simulink library "mssSimulink"  (R2024a)
settings: Solver=ode45  StartTime=0.0  StopTime=10.0  RelTol=1e-3
undefined symbols (not defined in the file): ABC, CN_data, CX_data, CY_data, D, G, Hoerner, K_supply, kt2ms, MA, magnitude, MRB, pathlength, RAO_Amp, RAO_Dir, RAO_Freq, RAO_Phase, RAO_Vel, RAO_yaw_back, RAO_yaw_quant, RAO_yaw_quantization_flag, rho_a, slcm, T_supply, table, vessel, vesselABC
libraries: $bdroot x99, simulink x13
(part 7 of 9)

== system mssSimulink/Modelling/Kinematics/Euler angles to rotation matrix ==
  theta : Inport
  Mux : Mux  Inputs=2
  Mux2 : Mux  Inputs=9
  R11 : Fcn  Expr=u(6)*u(5)
  R12 : Fcn  Expr=u(6)*u(2)*u(1)-u(3)*u(4)
  R13 : Fcn  Expr=u(4)*u(2)*u(6)+u(3)*u(1)
  "R21 " : Fcn  Expr=u(3)*u(5)
  R22 : Fcn  Expr=u(3)*u(2)*u(1)+u(6)*u(4)
  R23 : Fcn  Expr=u(3)*u(2)*u(4)-u(6)*u(1)
  "R31 " : Fcn  Expr=-u(2)
  R32 : Fcn  Expr=u(5)*u(1)
  R33 : Fcn  Expr=u(5)*u(4)
  Reshape 9x1->3x3 : Reshape  OutputDimensionality=Customize  OutputDimensions=[3,3]
  cos(theta) : Trigonometry  Operator=cos
  sin(theta) : Trigonometry
  Rzyx : Outport  InitialOutput=0  VectorParamsAs1DForOutWhenUnconnected=off
  wires:
  R11/1 -> Mux2/1
  Mux2/1 -> Reshape 9x1->3x3/1
  Reshape 9x1->3x3/1 -> Rzyx/1
  sin(theta)/1 -> Mux/1
  cos(theta)/1 -> Mux/2
  theta/1 -> sin(theta)/1, cos(theta)/1
  Mux/1 -> R32/1, R13/1, R33/1, R23/1, R22/1, "R31 "/1, R11/1, "R21 "/1, R12/1
  R23/1 -> Mux2/8
  R13/1 -> Mux2/7
  R22/1 -> Mux2/5
  R12/1 -> Mux2/4
  "R31 "/1 -> Mux2/3
  "R21 "/1 -> Mux2/2
  R32/1 -> Mux2/6
  R33/1 -> Mux2/9

== system mssSimulink/Modelling/Kinematics/Euler angles to attitude transformation matrix ==
  theta : Inport
  Constant : Constant
  "Constant " : Constant  Value=0
  Mux2 : Mux  Inputs=9
  Reshape 9x1->3x3 : Reshape  OutputDimensionality=Customize  OutputDimensions=[3,3]
  "T21 " : Fcn  Expr=sin(u(1))*tan(u(2))
  T22 : Fcn  Expr=cos(u(1))
  T23 : Fcn  Expr=sin(u(1))/cos(u(2))
  "T31 " : Fcn  Expr=cos(u(1))*tan(u(2))
  T32 : Fcn  Expr=-sin(u(1))
  T33 : Fcn  Expr=cos(u(1))/cos(u(2))
  T : Outport  InitialOutput=0  VectorParamsAs1DForOutWhenUnconnected=off
  wires:
  Constant/1 -> Mux2/1
  Mux2/1 -> Reshape 9x1->3x3/1
  Reshape 9x1->3x3/1 -> T/1
  theta/1 -> T23/1, T33/1, T32/1, "T31 "/1, T22/1, "T21 "/1
  T23/1 -> Mux2/6
  T22/1 -> Mux2/5
  T33/1 -> Mux2/9
  "Constant "/1 -> Mux2/2, Mux2/3
  "T21 "/1 -> Mux2/4
  "T31 "/1 -> Mux2/7
  T32/1 -> Mux2/8

== system mssSimulink/Modelling/Kinematics/Rotation matrix in yaw  ==
  psi : Inport
  nu : Inport  Port=2
  Fcn : Fcn  Expr=cos(u(1))*u(2)-sin(u(1))*u(3)
  Fcn1 : Fcn  Expr=sin(u(1))*u(2)+cos(u(1))*u(3)
  Fcn2 : Fcn  Expr=u(4)
  Mux : Mux  Inputs=2
  Mux1 : Mux  Inputs=3
  R*nu : Outport  VectorParamsAs1DForOutWhenUnconnected=off
  wires:
  Mux/1 -> Fcn2/1, Fcn1/1, Fcn/1
  Fcn/1 -> Mux1/1  "x_dot"
  Fcn1/1 -> Mux1/2  "y_dot"
  Fcn2/1 -> Mux1/3  "psi_dot"
  Mux1/1 -> R*nu/1  "eta_dot"
  psi/1 -> Mux/1
  nu/1 -> Mux/2

== system mssSimulink/Modelling/Kinematics/Transformation of generalized force ==
  tau : Inport
  r_p : Inport  Port=2
  Mux : Mux  Inputs=9
  Mux1 : Mux  Inputs=2
  Product : Product  Multiplication=Matrix(*)  SaturateOnIntegerOverflow=on  OutDataTypeStr=Inherit: Same as first input
  Reshape 9x1 => 3x3 : Reshape  OutputDimensionality=Customize  OutputDimensions=[3,3]
  Selector1 : Selector  InputPortWidth=6  IndexOptions=Index vector (dialog)  Indices=[4 5 6]  OutputSizes=1
  Selector2 : Selector  InputPortWidth=6  IndexOptions=Index vector (dialog)  Indices=[1 2 3]  OutputSizes=1
  Sum : Sum  SaturateOnIntegerOverflow=on
  h11 : Fcn  Expr=0
  h12 : Fcn  Expr=u(3)
  h13 : Fcn  Expr=-u(2)
  h21 : Fcn  Expr=-u(3)
  h22 : Fcn  Expr=0
  h23 : Fcn  Expr=u(1)
  h31 : Fcn  Expr=u(2)
  h32 : Fcn  Expr=-u(1)
  h33 : Fcn  Expr=0
  inv(H'(r_p))*tau : Outport  VectorParamsAs1DForOutWhenUnconnected=off
  wires:
  tau/1 -> Selector1/1, Selector2/1
  Selector1/1 -> Sum/2  "m"
  Mux/1 -> Reshape 9x1 => 3x3/1
  Reshape 9x1 => 3x3/1 -> Product/1  "S'(r_12)"
  h11/1 -> Mux/1
  h21/1 -> Mux/2
  h31/1 -> Mux/3
  h12/1 -> Mux/4
  h22/1 -> Mux/5
  h32/1 -> Mux/6
  h13/1 -> Mux/7
  h23/1 -> Mux/8
  h33/1 -> Mux/9
  r_p/1 -> h11/1, h21/1, h31/1, h12/1, h22/1, h32/1, h13/1, h23/1, h33/1
  Mux1/1 -> inv(H'(r_p))*tau/1
  Selector2/1 -> Mux1/1, Product/2  "f"
  Sum/1 -> Mux1/2
  Product/1 -> Sum/1

== system mssSimulink/Modelling/Kinematics/Transformation of generalized velocity ==
  note: S'(r_p)
  note: omega
  note: v
  nu : Inport
  r_p : Inport  Port=2
  Mux : Mux  Inputs=9
  Mux1 : Mux  Inputs=2
  Product : Product  Multiplication=Matrix(*)  SaturateOnIntegerOverflow=on  OutDataTypeStr=Inherit: Same as first input
  Reshape 9x1 => 3x3 : Reshape  OutputDimensionality=Customize  OutputDimensions=[3,3]
  Selector1 : Selector  InputPortWidth=6  IndexOptions=Index vector (dialog)  Indices=[4 5 6]  OutputSizes=1
  Selector2 : Selector  InputPortWidth=6  IndexOptions=Index vector (dialog)  Indices=[1 2 3]  OutputSizes=1
  Sum : Sum  SaturateOnIntegerOverflow=on
  h11 : Fcn  Expr=0
  h12 : Fcn  Expr=u(3)
  h13 : Fcn  Expr=-u(2)
  h21 : Fcn  Expr=-u(3)
  h22 : Fcn  Expr=0
  h23 : Fcn  Expr=u(1)
  h31 : Fcn  Expr=u(2)
  h32 : Fcn  Expr=-u(1)
  h33 : Fcn  Expr=0
  H(r_p)*nu : Outport  VectorParamsAs1DForOutWhenUnconnected=off
  wires:
  Selector2/1 -> Sum/2
  Product/1 -> Sum/1
  Selector1/1 -> Product/2, Mux1/2
  Sum/1 -> Mux1/1
  Mux1/1 -> H(r_p)*nu/1
  r_p/1 -> h33/1, h23/1, h13/1, h32/1, h22/1, h12/1, h31/1, h21/1, h11/1
  h33/1 -> Mux/9
  h23/1 -> Mux/8
  h13/1 -> Mux/7
  h32/1 -> Mux/6
  h22/1 -> Mux/5
  h12/1 -> Mux/4
  h31/1 -> Mux/3
  h21/1 -> Mux/2
  h11/1 -> Mux/1
  Reshape 9x1 => 3x3/1 -> Product/1
  Mux/1 -> Reshape 9x1 => 3x3/1
  nu/1 -> Selector2/1, Selector1/1

== system mssSimulink/Modelling/Kinematics/Transposed rotation matrix in yaw ==
  psi : Inport
  nu : Inport  Port=2
  Mux : Mux  Inputs=2
  Mux1 : Mux  Inputs=3
  Row1 : Fcn  Expr=cos(u(1))*u(2)+sin(u(1))*u(3)
  Row2 : Fcn  Expr=-sin(u(1))*u(2)+cos(u(1))*u(3)
  Row3 : Fcn  Expr=u(4)
  Out1 : Outport  VectorParamsAs1DForOutWhenUnconnected=off
  wires:
  nu/1 -> Mux/2
  psi/1 -> Mux/1
  Mux1/1 -> Out1/1
  Row3/1 -> Mux1/3
  Row2/1 -> Mux1/2
  Row1/1 -> Mux1/1
  Mux/1 -> Row1/1, Row2/1, Row3/1

== system mssSimulink/Modelling/Kinetics /3 DOF Eqs. of motion ==
  M_RB : Inport
  M_A : Inport  Port=2
  tau : Inport  Port=3
  nu_c : Inport  Port=4
  "0 or 1   " : Gain  Gain=CoriolisOnOff-1  SaturateOnIntegerOverflow=on  OutDataTypeStr=Inherit: Same as input  ParamDataTypeStr=Inherit: Same as input
  0-1 : Gain  Gain=CoriolisOnOff  SaturateOnIntegerOverflow=on  OutDataTypeStr=Inherit: Same as input  ParamDataTypeStr=Inherit: Same as input
  3 to 6 DOF : $bdroot/Modelling/Kinetics /Support/3 to 6 DOF  SystemSampleTime=-1  VariantActivationTime=update diagram  AllowFlexibleInterface=on  Latency=0  AutoFrameSizeCalculation=off
  3 to 6 DOF1 : $bdroot/Modelling/Kinetics /Support/3 to 6 DOF  SystemSampleTime=-1  VariantActivationTime=update diagram  AllowFlexibleInterface=on  Latency=0  AutoFrameSizeCalculation=off
  6 DOF Coriolis forces : $bdroot/Modelling/Kinetics /Support/6 DOF Coriolis forces  SystemSampleTime=-1  VariantActivationTime=update diagram  AllowFlexibleInterface=on  Latency=0  AutoFrameSizeCalculation=off
  6 DOF Coriolis forces1 : $bdroot/Modelling/Kinetics /Support/6 DOF Coriolis forces  SystemSampleTime=-1  VariantActivationTime=update diagram  AllowFlexibleInterface=on  Latency=0  AutoFrameSizeCalculation=off
  6 to 3 DOF : Selector  InputPortWidth=6  IndexOptions=Index vector (dialog)  Indices=[1 2 6]  OutputSizes=1
  6 to 3 DOF1 : Selector  InputPortWidth=6  IndexOptions=Index vector (dialog)  Indices=[1 2 6]  OutputSizes=1
  Integrator1 : Integrator  InitialCondition=nu0
  Integrator2 : Integrator  InitialCondition=eta0
  M33 to M66 : $bdroot/Modelling/Kinetics /Support/M33 to M66  SystemSampleTime=-1  VariantActivationTime=update diagram  AllowFlexibleInterface=on  Latency=0  AutoFrameSizeCalculation=off
  M33 to M661 : $bdroot/Models/ Kinetics /Support/M33 to M66
  Product : Product  Inputs=/*  Multiplication=Matrix(*)  SaturateOnIntegerOverflow=on  OutDataTypeStr=Inherit: Same as first input
  "Rotation matrix in yaw " : $bdroot/Modelling/Kinematics/Rotation matrix in yaw 
  Selector2 : Selector  InputPortWidth=3  IndexOptions=Index vector (dialog)  Indices=[3]  OutputSizes=1
  Sum : Sum  Inputs=|+-  SaturateOnIntegerOverflow=on
  Sum1 : Sum  Inputs=|+-  SaturateOnIntegerOverflow=on
  Sum2 : Sum  SaturateOnIntegerOverflow=on
  Sum3 : Sum  Inputs=|+-  SaturateOnIntegerOverflow=on
  eta : Outport  VectorParamsAs1DForOutWhenUnconnected=off
  nu : Outport  Port=2  VectorParamsAs1DForOutWhenUnconnected=off
  wires:
  6 to 3 DOF1/1 -> Sum3/2
  6 to 3 DOF/1 -> Sum/2  "C_RB(nu)nu"
  6 DOF Coriolis forces1/1 -> 6 to 3 DOF1/1  "C_A(nu_r)nu_r"
  Sum3/1 -> Product/2
  Sum/1 -> Sum3/1
  3 to 6 DOF1/1 -> 6 DOF Coriolis forces1/2
  M33 to M66/1 -> 6 DOF Coriolis forces1/1
  M_A/1 -> Sum2/1, M33 to M66/1  "M_A"
  nu_c/1 -> Sum1/2
  Sum1/1 -> "0 or 1   "/1
  "0 or 1   "/1 -> 3 to 6 DOF1/1  "nu_r"
  Sum2/1 -> Product/1
  M_RB/1 -> Sum2/2, M33 to M661/1
  Integrator1/1 -> 0-1/1, Sum1/1, nu/1, "Rotation matrix in yaw "/2  "nu"
  M33 to M661/1 -> 6 DOF Coriolis forces/1
  6 DOF Coriolis forces/1 -> 6 to 3 DOF/1
  3 to 6 DOF/1 -> 6 DOF Coriolis forces/2
  0-1/1 -> 3 to 6 DOF/1
  tau/1 -> Sum/1
  Selector2/1 -> "Rotation matrix in yaw "/1  "psi"
  Integrator2/1 -> eta/1, Selector2/1  "eta"
  "Rotation matrix in yaw "/1 -> Integrator2/1  "d(eta)/dt"
  Product/1 -> Integrator1/1  "d(nu)/dt"

== system mssSimulink/Modelling/Kinetics /6 DOF Eqs. of motion ==
  M_RB : Inport
  M_A : Inport  Port=2
  tau : Inport  Port=3
  nu_c : Inport  Port=4
  0 or 1 : Gain  Gain=CoriolisOnOff-1  SaturateOnIntegerOverflow=on  OutDataTypeStr=Inherit: Same as input  ParamDataTypeStr=Inherit: Same as input
  "0 or 1   " : Gain  Gain=CoriolisOnOff-1  SaturateOnIntegerOverflow=on  OutDataTypeStr=Inherit: Same as input  ParamDataTypeStr=Inherit: Same as input
  6 DOF Coriolis forces : $bdroot/Modelling/Kinetics /Support/6 DOF Coriolis forces  SystemSampleTime=-1  VariantActivationTime=update diagram  AllowFlexibleInterface=on  Latency=0  AutoFrameSizeCalculation=off
  6 DOF Coriolis forces1 : $bdroot/Modelling/Kinetics /Support/6 DOF Coriolis forces  SystemSampleTime=-1  VariantActivationTime=update diagram  AllowFlexibleInterface=on  Latency=0  AutoFrameSizeCalculation=off
  Euler angles to rotation matrix : $bdroot/Modelling/Kinematics/Euler angles to rotation matrix
  Euler angles to attitude transformation matrix : $bdroot/Modelling/Kinematics/Euler angles to attitude transformation matrix
  Integrator : Integrator  InitialCondition=nu0
  Integrator1 : Integrator  InitialCondition=eta0(1:3)
  Integrator2 : Integrator  InitialCondition=eta0(4:6)
  Mux : Mux  Inputs=2
  Mux1 : Mux  Inputs=2
  Product : Product  Inputs=/*  Multiplication=Matrix(*)  SaturateOnIntegerOverflow=on  OutDataTypeStr=Inherit: Same as first input
  Product1 : Product  Inputs=**  Multiplication=Matrix(*)  SaturateOnIntegerOverflow=on  OutDataTypeStr=Inherit: Same as first input
  Product2 : Product  Inputs=**  Multiplication=Matrix(*)  SaturateOnIntegerOverflow=on  OutDataTypeStr=Inherit: Same as first input
  Selector1 : Selector  InputPortWidth=6  IndexOptions=Index vector (dialog)  Indices=[1 2 3]  OutputSizes=1
  Selector2 : Selector  InputPortWidth=6  IndexOptions=Index vector (dialog)  Indices=[4 5 6]  OutputSizes=1
  Sum : Sum  Inputs=|+-  SaturateOnIntegerOverflow=on
  Sum1 : Sum  Inputs=|+-  SaturateOnIntegerOverflow=on
  Sum2 : Sum  SaturateOnIntegerOverflow=on
  Sum3 : Sum  Inputs=|+-  SaturateOnIntegerOverflow=on
  eta : Outport  VectorParamsAs1DForOutWhenUnconnected=off
  nu : Outport  Port=2  VectorParamsAs1DForOutWhenUnconnected=off
  wires:
  nu_c/1 -> Sum1/2
  Sum1/1 -> "0 or 1   "/1
  "0 or 1   "/1 -> 6 DOF Coriolis forces1/2  "nu_r"
  6 DOF Coriolis forces1/1 -> Sum3/2  "C_A(nu_r)nu_r"
  Sum3/1 -> Product/2
  Sum/1 -> Sum3/1
  Sum2/1 -> Product/1  "M"
  M_A/1 -> Sum2/1, 6 DOF Coriolis forces1/1  "M_A"
  M_RB/1 -> Sum2/2, 6 DOF Coriolis forces/1  "M_RB"
  Product/1 -> Integrator/1  "(d/dt)nu"
  Integrator/1 -> Selector1/1, Selector2/1, 0 or 1/1  "nu"
  Selector1/1 -> Product1/2, Mux1/1  "v"
  Selector2/1 -> Mux1/2, Product2/2  "w_nb"
  Product1/1 -> Integrator1/1  "dp/dt"
  Euler angles to rotation matrix/1 -> Product1/1  "R(theta)"
  Product2/1 -> Integrator2/1  "(d/dt)theta"
  Integrator2/1 -> Mux/2, Euler angles to rotation matrix/1, Euler angles to attitude transformation matrix/1  "theta"
  Integrator1/1 -> Mux/1  "p"
  Mux/1 -> eta/1  "eta"
  Mux1/1 -> Sum1/1, nu/1  "nu"
  Euler angles to attitude transformation matrix/1 -> Product2/1
  tau/1 -> Sum/1
  6 DOF Coriolis forces/1 -> Sum/2  "C_RB(nu)nu"
  0 or 1/1 -> 6 DOF Coriolis forces/2

== system mssSimulink/Modelling/Kinetics /Support ==
  3 to 6 DOF : Subsystem
      mask Display: disp('modes,\n 1,2,6, to\n 6 DOF')
  4 to 6 DOF : Subsystem
      mask Display: disp('modes,\n 1,2,4,6, to\n 6 DOF')
  6 DOF Coriolis forces : Subsystem
  6 to 3 DOF : Selector  InputPortWidth=6  IndexOptions=Index vector (dialog)  Indices=[1 2 6]  OutputSizes=1
  6 to 4 DOF : Selector  InputPortWidth=6  IndexOptions=Index vector (dialog)  Indices=[1 2 4 6]  OutputSizes=1
  M33 to M66 : Subsystem
      mask Display: disp('add zeros')
  M44 to M66 : Subsystem
      mask Display: disp('add zeros')
  M66 to M33 : Selector  NumberOfDimensions=2  InputPortWidth=3  IndexOptions=Index vector (dialog),Index vector (dialog)  Indices=[1 2 6],[1 2 6]  OutputSizes=1
  M66 to M44 : Selector  NumberOfDimensions=2  InputPortWidth=3  IndexOptions=Index vector (dialog),Index vector (dialog)  Indices=[1 2 4 6],[1 2 4 6]  OutputSizes=1

== system mssSimulink/Modelling/Propulsion/Actuator Configuration ==
  2 main propellers and 3 tunnel  thrusters : Subsystem
      mask Display: disp('tau = T*K(n)*u')
  "2 main propellers, 1 azimuth and 2 tunnel thrusters" : Subsystem
      mask Display:
      | disp('tau =            \n\n')
      | disp('    T(alpha)*K(n)*u')
  4 azimuth thrusters : Subsystem
      mask Display:
      | disp('tau =            \n\n')
      | disp('    T(alpha)*K(n)*u')
  Column vector t : Subsystem
  Thruster configuration matrix : Subsystem

== system mssSimulink/Modelling/Propulsion/Open-water propeller characteristics ==
  n : Inport
  Va : Inport  Port=2
  Dot Product1 : DotProduct  OutDataTypeStr=Inherit: Inherit via internal rule
  Dot Product2 : DotProduct  OutDataTypeStr=Inherit: Inherit via internal rule
  Kq poly : Constant  Value=Par_Thruster_Kqp
  Kt poly : Constant  Value=Par_Thruster_Ktp
  Math Function3 : Math  Operator=magnitude^2  SignedPower=on
  Math Function4 : Math  Operator=magnitude^2  SignedPower=on
  Mux1 : Mux  Inputs=3
  Product{2..3,6,9..10} (5 alike) : Product  SaturateOnIntegerOverflow=on  OutDataTypeStr=Inherit: Same as first input
  Sign : Signum
  Switch : Switch  InputSameDT=off
  Zero limit : Saturate  UpperLimit=inf  LowerLimit=0
  Zero limit1 : Saturate  UpperLimit=inf  LowerLimit=0
  Zero limit2 : Saturate  UpperLimit=inf  LowerLimit=0
  reverse reduction : Gain  Gain=Par_Thruster_reverse_reduction  SaturateOnIntegerOverflow=on  OutDataTypeStr=Inherit: Same as input  ParamDataTypeStr=Inherit: Same as input
  rhow[D^2 D^3 D^4] : Constant  Value=Glob_rhow*[Par_Thruster_D^2 Par_Thruster_D^3 Par_Thruster_D^4]
  "rhow[D^3 D^4 D^5] " : Constant  Value=Glob_rhow*[Par_Thruster_D^3 Par_Thruster_D^4 Par_Thruster_D^5]
  T_a : Outport  VectorParamsAs1DForOutWhenUnconnected=off
  Q_a : Outport  Port=2  VectorParamsAs1DForOutWhenUnconnected=off
  wires:
  Product10/1 -> Mux1/2
  Math Function4/1 -> Mux1/3
  Math Function3/1 -> Mux1/1
  n/1 -> Sign/1, Product10/2, Math Function4/1
  Product9/1 -> Dot Product2/2
  "rhow[D^3 D^4 D^5] "/1 -> Product9/2
  Kq poly/1 -> Product9/1
  Product6/1 -> Dot Product1/1
  rhow[D^2 D^3 D^4]/1 -> Product6/2
  Kt poly/1 -> Product6/1
  Sign/1 -> Product3/2, Switch/2, Product2/2
  Va/1 -> Zero limit2/1
  Zero limit1/1 -> Product3/1
  Zero limit/1 -> Product2/1
  Dot Product2/1 -> Zero limit1/1
  Dot Product1/1 -> Zero limit/1
  Product3/1 -> Q_a/1
  Product2/1 -> Switch/1, reverse reduction/1
  Switch/1 -> T_a/1
  reverse reduction/1 -> Switch/3
  Mux1/1 -> Dot Product2/1, Dot Product1/2
  Zero limit2/1 -> Math Function3/1, Product10/1

== system mssSimulink/Modelling/Propulsion/Propeller shaft dynamics ==
  RPM_c : Inport
  Gain : Gain  Gain=1/tc  SaturateOnIntegerOverflow=on  OutDataTypeStr=Inherit: Same as input  ParamDataTypeStr=Inherit: Same as input
  Integrator1 : Integrator
  Saturation : Saturate  UpperLimit=rpm_rate  LowerLimit=-rpm_rate
  Saturation1 : Saturate  UpperLimit=rpm_max  LowerLimit=-rpm_max
  Sum1 : Sum  Inputs=|+-  InputSameDT=on  SaturateOnIntegerOverflow=on  OutDataTypeStr=Inherit: Same as first input
  RPM : Outport  VectorParamsAs1DForOutWhenUnconnected=off
  wires:
  RPM_c/1 -> Saturation1/1
  Saturation/1 -> Integrator1/1
  Saturation1/1 -> Sum1/1
  Integrator1/1 -> Sum1/2, RPM/1
  Sum1/1 -> Gain/1
  Gain/1 -> Saturation/1

== system mssSimulink/Navigation/Estimators/Discerte-time EKF for SOG and COG ==
  xpos : Inport
  ypos : Inport  Port=2
  Five-state EKF for North-East positions : MATLAB Function  InitFcn=clear EKF_5states;  TreatAsAtomicUnit=on
  Qd : Constant  Value=Qd
  RT : RateTransition  OutPortSampleTime=0
  Rate Transition : RateTransition  OutPortSampleTimeMultiple=10  OutPortSampleTime=h_samp
  Rate Transition1 : RateTransition  OutPortSampleTimeMultiple=10  OutPortSampleTime=h_samp
  Rd : Constant  Value=Rd
  alpha_1 : Constant  Value=alpha_1
  alpha_2 : Constant  Value=alpha_2
  h_samp : Constant  Value=h_samp
  x_hat : Outport
  wires:
  RT/1 -> x_hat/1
  xpos/1 -> Rate Transition/1
  ypos/1 -> Rate Transition1/1
  h_samp/1 -> Five-state EKF for North-East positions/3(h_samp)
  Five-state EKF for North-East positions/1(x_hat) -> RT/1
  Rate Transition/1 -> Five-state EKF for North-East positions/1(position1)
  Rate Transition1/1 -> Five-state EKF for North-East positions/2(position2)
  Qd/1 -> Five-state EKF for North-East positions/4(Qd)
  Rd/1 -> Five-state EKF for North-East positions/5(Rd)
  alpha_1/1 -> Five-state EKF for North-East positions/6(alpha_1)
  alpha_2/1 -> Five-state EKF for North-East positions/7(alpha_2)

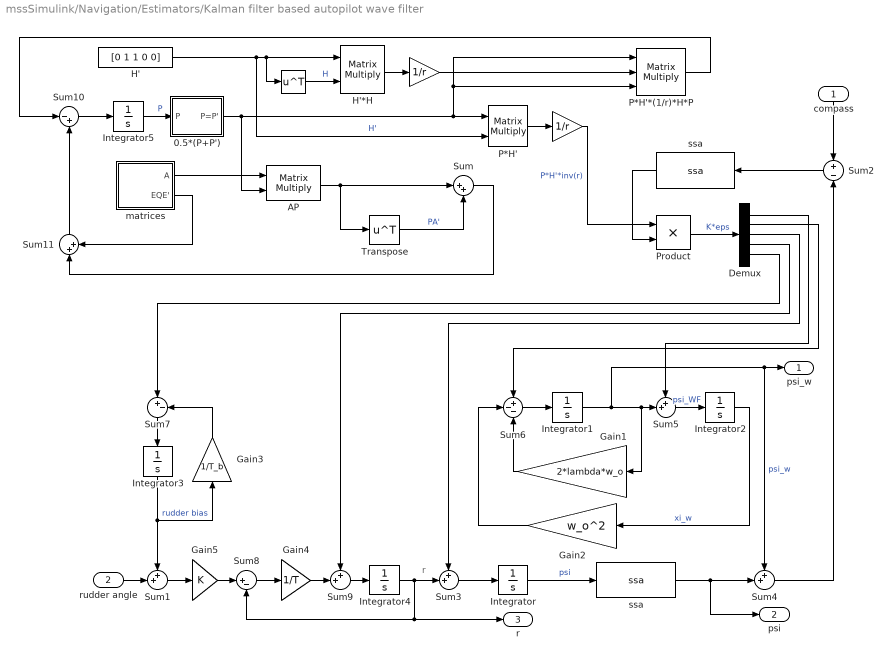
== system mssSimulink/Navigation/Estimators/Kalman filter based autopilot wave filter ==
  note: r
  compass : Inport
  rudder angle : Inport  Port=2
  "  " : Math  Operator=transpose  SignedPower=on
  "    " : Gain  Gain=1/r  SaturateOnIntegerOverflow=on  OutDataTypeStr=Inherit: Same as input  ParamDataTypeStr=Inherit: Same as input
  "     " : Gain  Gain=1/r  SaturateOnIntegerOverflow=on  OutDataTypeStr=Inherit: Same as input  ParamDataTypeStr=Inherit: Same as input
  0.5*(P+P') : Subsystem
  AP : Product  Multiplication=Matrix(*)  SaturateOnIntegerOverflow=on  OutDataTypeStr=Inherit: Same as first input
  Demux : Demux  Outputs=5
      settings: DisplayOption=none
  Gain1 : Gain  Gain=2*lambda*w_o  SaturateOnIntegerOverflow=on  OutDataTypeStr=Inherit: Same as input  ParamDataTypeStr=Inherit: Same as input
  Gain2 : Gain  Gain=w_o^2  SaturateOnIntegerOverflow=on  OutDataTypeStr=Inherit: Same as input  ParamDataTypeStr=Inherit: Same as input
  Gain3 : Gain  Gain=1/T_b  SaturateOnIntegerOverflow=on  OutDataTypeStr=Inherit: Same as input  ParamDataTypeStr=Inherit: Same as input
  Gain4 : Gain  Gain=1/T  SaturateOnIntegerOverflow=on  OutDataTypeStr=Inherit: Same as input  ParamDataTypeStr=Inherit: Same as input
  Gain5 : Gain  Gain=K  SaturateOnIntegerOverflow=on  OutDataTypeStr=Inherit: Same as input  ParamDataTypeStr=Inherit: Same as input
  H' : Constant  Value=[0 1 1 0 0]
  H'*H : Product  Multiplication=Matrix(*)  SaturateOnIntegerOverflow=on  OutDataTypeStr=Inherit: Same as first input
  Integrator{,1..4} (5 alike) : Integrator
  Integrator5 : Integrator  InitialCondition=P0
  P*H' : Product  Inputs=**  Multiplication=Matrix(*)  SaturateOnIntegerOverflow=on  OutDataTypeStr=Inherit: Same as first input
  P*H'*(1/r)*H*P : Product  Inputs=***  Multiplication=Matrix(*)  SaturateOnIntegerOverflow=on  OutDataTypeStr=Inherit: Same as first input
  Product : Product  SaturateOnIntegerOverflow=on  OutDataTypeStr=Inherit: Same as first input
  Sum : Sum  Inputs=|++  SaturateOnIntegerOverflow=on
  Sum{1,3..5,9} (5 alike) : Sum  Inputs=++|  InputSameDT=on  SaturateOnIntegerOverflow=on  OutDataTypeStr=Inherit: Same as first input
  Sum10 : Sum  Inputs=|-+  SaturateOnIntegerOverflow=on
  Sum11 : Sum  Inputs=|++  SaturateOnIntegerOverflow=on
  Sum2 : Sum  Inputs=+|-  InputSameDT=on  SaturateOnIntegerOverflow=on  OutDataTypeStr=Inherit: Same as first input
  Sum6 : Sum  Inputs=+--  InputSameDT=on  SaturateOnIntegerOverflow=on  OutDataTypeStr=Inherit: Same as first input
  Sum7 : Sum  Inputs=|+-  InputSameDT=on  SaturateOnIntegerOverflow=on  OutDataTypeStr=Inherit: Same as first input
  Sum8 : Sum  Inputs=|+-  InputSameDT=on  SaturateOnIntegerOverflow=on  OutDataTypeStr=Inherit: Same as first input
  Transpose : Math  Operator=transpose  SignedPower=on
  matrices : Subsystem
  "ssa " : $bdroot/Utilities/Math Operations/ssa  SystemSampleTime=-1  VariantActivationTime=update diagram  AllowFlexibleInterface=on  Latency=0  AutoFrameSizeCalculation=off
  "ssa  " : $bdroot/Utilities/Math Operations/ssa  SystemSampleTime=-1  VariantActivationTime=update diagram  AllowFlexibleInterface=on  Latency=0  AutoFrameSizeCalculation=off
  psi_w : Outport  VectorParamsAs1DForOutWhenUnconnected=off
  psi : Outport  Port=2  VectorParamsAs1DForOutWhenUnconnected=off
  r : Outport  Port=3  VectorParamsAs1DForOutWhenUnconnected=off
  wires:
  0.5*(P+P')/1(P=P') -> P*H'*(1/r)*H*P/1, P*H'*(1/r)*H*P/3, P*H'/1, AP/2
  Integrator5/1 -> 0.5*(P+P')/1(P)  "P"
  P*H'*(1/r)*H*P/1 -> Sum10/1
  Demux/4 -> Sum9/1
  Demux/3 -> Sum3/1
  Demux/2 -> Sum6/1
  Demux/1 -> Sum5/1
  Product/1 -> Demux/1  "K*eps"
  "ssa "/1 -> Product/2
  Sum/1 -> Sum11/1
  matrices/2(EQE') -> Sum11/2
  "     "/1 -> Product/1  "P*H'*inv(r)"
  Sum11/1 -> Sum10/2
  Transpose/1 -> Sum/2  "PA'"
  Sum10/1 -> Integrator5/1
  AP/1 -> Transpose/1, Sum/1
  Sum9/1 -> Integrator4/1
  Gain4/1 -> Sum9/2
  Gain5/1 -> Sum8/1
  Gain3/1 -> Sum7/2
  Integrator3/1 -> Gain3/1, Sum1/1  "rudder bias"
  Sum7/1 -> Integrator3/1
  Demux/5 -> Sum7/1
  Integrator4/1 -> Sum3/2, r/1, Sum8/2
  Sum8/1 -> Gain4/1
  rudder angle/1 -> Sum1/2
  compass/1 -> Sum2/1
  Sum1/1 -> Gain5/1
  Integrator1/1 -> psi_w/1, Sum4/1, Gain1/1, Sum5/2  "psi_w"
  Sum5/1 -> Integrator2/1  "psi_WF"
  Integrator2/1 -> Gain2/1  "xi_w"
  Gain2/1 -> Sum6/2
  Gain1/1 -> Sum6/3
  Sum6/1 -> Integrator1/1
  Sum4/1 -> Sum2/2
  "ssa  "/1 -> psi/1, Sum4/2
  Integrator/1 -> "ssa  "/1  "psi"
  Sum2/1 -> "ssa "/1
  Sum3/1 -> Integrator/1
  H'/1 -> "  "/1, H'*H/1, P*H'/2  "H'"
  H'*H/1 -> "    "/1
  P*H'/1 -> "     "/1
  "    "/1 -> P*H'*(1/r)*H*P/2
  "  "/1 -> H'*H/2  "H"
  matrices/1(A) -> AP/1

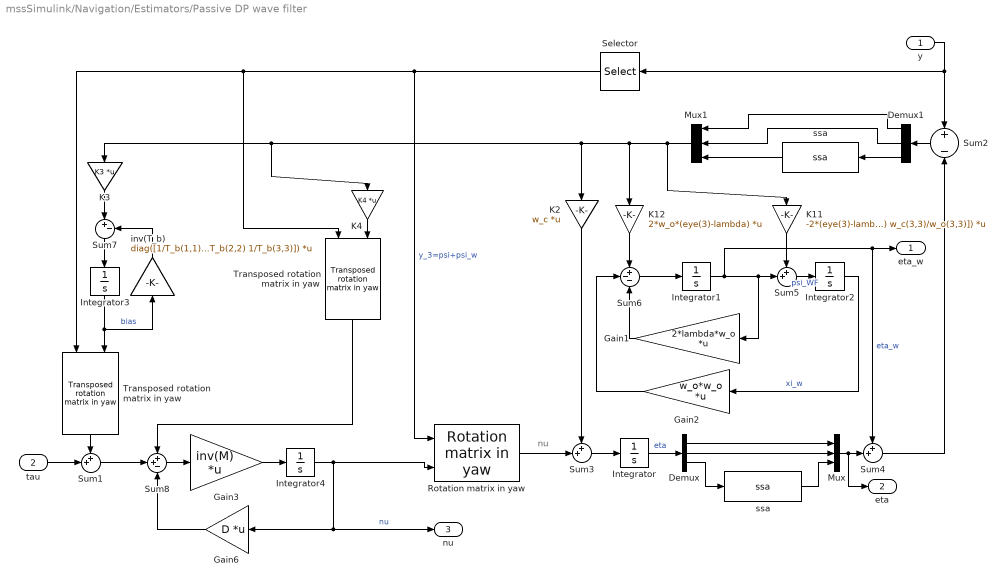
== system mssSimulink/Navigation/Estimators/Passive DP wave filter ==
  note: nu
  y : Inport
  tau : Inport  Port=2
  Demux : Demux  Outputs=3
      settings: DisplayOption=none
  Demux1 : Demux  Outputs=3
      settings: DisplayOption=none
  Gain1 : Gain  Gain=2*lambda*w_o  Multiplication=Matrix(K*u)  SaturateOnIntegerOverflow=on  OutDataTypeStr=Inherit: Same as input  ParamDataTypeStr=Inherit: Same as input
  Gain2 : Gain  Gain=w_o*w_o  Multiplication=Matrix(K*u)  SaturateOnIntegerOverflow=on  OutDataTypeStr=Inherit: Same as input  ParamDataTypeStr=Inherit: Same as input
  Gain3 : Gain  Gain=inv(M)  Multiplication=Matrix(K*u)  SaturateOnIntegerOverflow=on  OutDataTypeStr=Inherit: Same as input  ParamDataTypeStr=Inherit: Same as input
  Gain6 : Gain  Gain=D  Multiplication=Matrix(K*u)  SaturateOnIntegerOverflow=on  OutDataTypeStr=Inherit: Same as input  ParamDataTypeStr=Inherit: Same as input
  Integrator{,1..4} (5 alike) : Integrator
  K11 : Gain  Gain=-2*(eye(3)-lambda)*diag([w_c(1,1)/w_o(1,1) w_c(2,2)/w_o(2,2) w_c(3,3)/w_o(3,3)])  Multiplication=Matrix(K*u)  SaturateOnIntegerOverflow=on  OutDataTypeStr=Inherit: Same as input  ParamDataTypeStr=Inherit: Same as input
  K12 : Gain  Gain=2*w_o*(eye(3)-lambda)  Multiplication=Matrix(K*u)  SaturateOnIntegerOverflow=on  OutDataTypeStr=Inherit: Same as input  ParamDataTypeStr=Inherit: Same as input
  K2 : Gain  Gain=w_c  Multiplication=Matrix(K*u)  SaturateOnIntegerOverflow=on  OutDataTypeStr=Inherit: Same as input  ParamDataTypeStr=Inherit: Same as input
  K3 : Gain  Gain=K3  Multiplication=Matrix(K*u)  SaturateOnIntegerOverflow=on  OutDataTypeStr=Inherit: Same as input  ParamDataTypeStr=Inherit: Same as input
  K4 : Gain  Gain=K4  Multiplication=Matrix(K*u)  SaturateOnIntegerOverflow=on  OutDataTypeStr=Inherit: Same as input  ParamDataTypeStr=Inherit: Same as input
  Mux : Mux  Inputs=3
  Mux1 : Mux  Inputs=3
  "Rotation matrix in yaw   " : $bdroot/Modelling/Kinematics/Rotation matrix in yaw 
  Selector : Selector  InputPortWidth=3  IndexOptions=Index vector (dialog)  Indices=[3]  OutputSizes=1
  Sum{1,3..5} (4 alike) : Sum  Inputs=++|  InputSameDT=on  SaturateOnIntegerOverflow=on  OutDataTypeStr=Inherit: Same as first input
  Sum2 : Sum  Inputs=+|-  InputSameDT=on  SaturateOnIntegerOverflow=on  OutDataTypeStr=Inherit: Same as first input
  Sum6 : Sum  Inputs=+--  InputSameDT=on  SaturateOnIntegerOverflow=on  OutDataTypeStr=Inherit: Same as first input
  Sum7 : Sum  Inputs=|+-  InputSameDT=on  SaturateOnIntegerOverflow=on  OutDataTypeStr=Inherit: Same as first input
  Sum8 : Sum  Inputs=++-  InputSameDT=on  SaturateOnIntegerOverflow=on  OutDataTypeStr=Inherit: Same as first input
  "Transposed rotation matrix in yaw " : $bdroot/Modelling/Kinematics/Transposed rotation  matrix in yaw
  "Transposed rotation matrix in yaw     " : $bdroot/Modelling/Kinematics/Transposed rotation  matrix in yaw
  inv(T_b) : Gain  Gain=diag([1/T_b(1,1) 1/T_b(2,2) 1/T_b(3,3)])  Multiplication=Matrix(K*u)  SaturateOnIntegerOverflow=on  OutDataTypeStr=Inherit: Same as input  ParamDataTypeStr=Inherit: Same as input
  "ssa " : $bdroot/Utilities/Math Operations/ssa  SystemSampleTime=-1  VariantActivationTime=update diagram  AllowFlexibleInterface=on  Latency=0  AutoFrameSizeCalculation=off
  "ssa   " : $bdroot/Utilities/Math Operations/ssa  SystemSampleTime=-1  VariantActivationTime=update diagram  AllowFlexibleInterface=on  Latency=0  AutoFrameSizeCalculation=off
  eta_w : Outport  VectorParamsAs1DForOutWhenUnconnected=off
  eta : Outport  Port=2  VectorParamsAs1DForOutWhenUnconnected=off
  nu : Outport  Port=3  VectorParamsAs1DForOutWhenUnconnected=off
  wires:
  Sum3/1 -> Integrator/1
  Mux1/1 -> K11/1, K12/1, K2/1, K3/1, K4/1
  Sum4/1 -> Sum2/2
  K2/1 -> Sum3/1
  Sum6/1 -> Integrator1/1
  Gain1/1 -> Sum6/3
  Gain2/1 -> Sum6/2
  Integrator2/1 -> Gain2/1  "xi_w"
  K11/1 -> Sum5/1
  K12/1 -> Sum6/1
  Sum5/1 -> Integrator2/1  "psi_WF"
  Integrator1/1 -> Sum5/2, Gain1/1, Sum4/1, eta_w/1  "eta_w"
  y/1 -> Sum2/1, Selector/1
  tau/1 -> Sum1/2
  Sum7/1 -> Integrator3/1
  Integrator3/1 -> inv(T_b)/1, "Transposed rotation matrix in yaw "/2  "bias"
  inv(T_b)/1 -> Sum7/2
  Integrator/1 -> Demux/1  "eta"
  "ssa "/1 -> Mux/3
  Mux/1 -> Sum4/2, eta/1
  Demux/1 -> Mux/1
  Demux/2 -> Mux/2
  "ssa   "/1 -> Mux1/3
  Demux1/2 -> Mux1/2
  Demux1/3 -> "ssa   "/1
  Sum2/1 -> Demux1/1
  Demux1/1 -> Mux1/1
  Selector/1 -> "Transposed rotation matrix in yaw     "/1, "Transposed rotation matrix in yaw "/1, "Rotation matrix in yaw   "/1  "y_3=psi+psi_w"
  K4/1 -> "Transposed rotation matrix in yaw     "/2
  "Transposed rotation matrix in yaw     "/1 -> Sum8/1
  "Transposed rotation matrix in yaw "/1 -> Sum1/1
  K3/1 -> Sum7/1
  Integrator4/1 -> Gain6/1, nu/1, "Rotation matrix in yaw   "/2  "nu"
  "Rotation matrix in yaw   "/1 -> Sum3/2
  Gain3/1 -> Integrator4/1
  Sum1/1 -> Sum8/2
  Sum8/1 -> Gain3/1
  Gain6/1 -> Sum8/3
  Demux/3 -> "ssa "/1

== system mssSimulink/Navigation/Estimators/Passive autopilot wave filter 1 ==
  note: r
  compass : Inport
  rudder angle : Inport  Port=2
  Gain1 : Gain  Gain=2*lambda*w_o  SaturateOnIntegerOverflow=on  OutDataTypeStr=Inherit: Same as input  ParamDataTypeStr=Inherit: Same as input
  Gain2 : Gain  Gain=w_o^2  SaturateOnIntegerOverflow=on  OutDataTypeStr=Inherit: Same as input  ParamDataTypeStr=Inherit: Same as input
  Gain3 : Gain  Gain=1/T_b  SaturateOnIntegerOverflow=on  OutDataTypeStr=Inherit: Same as input  ParamDataTypeStr=Inherit: Same as input
  Gain4 : Gain  Gain=1/T  SaturateOnIntegerOverflow=on  OutDataTypeStr=Inherit: Same as input  ParamDataTypeStr=Inherit: Same as input
  Gain5 : Gain  Gain=K  SaturateOnIntegerOverflow=on  OutDataTypeStr=Inherit: Same as input  ParamDataTypeStr=Inherit: Same as input
  Integrator{,1..4} (5 alike) : Integrator
  K1 : Gain  Gain=-2*w_c*(1.0-lambda)/w_o  SaturateOnIntegerOverflow=on  OutDataTypeStr=Inherit: Same as input  ParamDataTypeStr=Inherit: Same as input
  K2 : Gain  Gain=2*w_o*(1.0-lambda)  SaturateOnIntegerOverflow=on  OutDataTypeStr=Inherit: Same as input  ParamDataTypeStr=Inherit: Same as input
  K3 : Gain  Gain=w_c  SaturateOnIntegerOverflow=on  OutDataTypeStr=Inherit: Same as input  ParamDataTypeStr=Inherit: Same as input
  K4 : Gain  Gain=K4  SaturateOnIntegerOverflow=on  OutDataTypeStr=Inherit: Same as input  ParamDataTypeStr=Inherit: Same as input
  K5 : Gain  Gain=K5  SaturateOnIntegerOverflow=on  OutDataTypeStr=Inherit: Same as input  ParamDataTypeStr=Inherit: Same as input
  Sum1 : Sum  Inputs=-+|  InputSameDT=on  SaturateOnIntegerOverflow=on  OutDataTypeStr=Inherit: Same as first input
  Sum2 : Sum  Inputs=+|-  InputSameDT=on  SaturateOnIntegerOverflow=on  OutDataTypeStr=Inherit: Same as first input
  Sum{3..5,9} (4 alike) : Sum  Inputs=++|  InputSameDT=on  SaturateOnIntegerOverflow=on  OutDataTypeStr=Inherit: Same as first input
  Sum6 : Sum  Inputs=+--  InputSameDT=on  SaturateOnIntegerOverflow=on  OutDataTypeStr=Inherit: Same as first input
  Sum7 : Sum  Inputs=|+-  InputSameDT=on  SaturateOnIntegerOverflow=on  OutDataTypeStr=Inherit: Same as first input
  Sum8 : Sum  Inputs=|+-  InputSameDT=on  SaturateOnIntegerOverflow=on  OutDataTypeStr=Inherit: Same as first input
  "ssa " : $bdroot/Utilities/Math Operations/ssa  SystemSampleTime=-1  VariantActivationTime=update diagram  AllowFlexibleInterface=on  Latency=0  AutoFrameSizeCalculation=off
  "ssa  " : $bdroot/Utilities/Math Operations/ssa  SystemSampleTime=-1  VariantActivationTime=update diagram  AllowFlexibleInterface=on  Latency=0  AutoFrameSizeCalculation=off
  psi_w : Outport  VectorParamsAs1DForOutWhenUnconnected=off
  psi : Outport  Port=2  VectorParamsAs1DForOutWhenUnconnected=off
  r : Outport  Port=3  VectorParamsAs1DForOutWhenUnconnected=off
  wires:
  Sum3/1 -> Integrator/1
  Sum2/1 -> "ssa  "/1
  "ssa  "/1 -> K1/1, K2/1, K3/1, K4/1, K5/1
  Integrator/1 -> "ssa "/1  "psi"
  "ssa "/1 -> psi/1, Sum4/2
  Sum4/1 -> Sum2/2
  K3/1 -> Sum3/1
  Sum6/1 -> Integrator1/1
  Gain1/1 -> Sum6/3
  Gain2/1 -> Sum6/2
  Integrator2/1 -> Gain2/1  "xi_w"
  K1/1 -> Sum5/1
  K2/1 -> Sum6/1
  Sum5/1 -> Integrator2/1  "psi_WF"
  Integrator1/1 -> Sum5/2, Gain1/1, Sum4/1, psi_w/1  "psi_w"
  Sum1/1 -> Gain5/1
  compass/1 -> Sum2/1
  rudder angle/1 -> Sum1/2
  Sum8/1 -> Gain4/1
  Integrator4/1 -> Sum8/2, r/1, Sum3/2
  K5/1 -> Sum7/1
  Sum7/1 -> Integrator3/1
  Integrator3/1 -> Sum1/1, Gain3/1  "rudder bias"
  Gain3/1 -> Sum7/2
  Gain5/1 -> Sum8/1
  Gain4/1 -> Sum9/2
  Sum9/1 -> Integrator4/1
  K4/1 -> Sum9/1

== system mssSimulink/Navigation/Estimators/Passive autopilot wave filter 2 ==
  compass : Inport
  rate gyro : Inport  Port=2
  Gain1 : Gain  Gain=2*lambda*w_o  SaturateOnIntegerOverflow=on  OutDataTypeStr=Inherit: Same as input  ParamDataTypeStr=Inherit: Same as input
  Gain2 : Gain  Gain=w_o^2  SaturateOnIntegerOverflow=on  OutDataTypeStr=Inherit: Same as input  ParamDataTypeStr=Inherit: Same as input
  Gain3 : Gain  Gain=1/T_b  SaturateOnIntegerOverflow=on  OutDataTypeStr=Inherit: Same as input  ParamDataTypeStr=Inherit: Same as input
  Integrator{,1..3} (4 alike) : Integrator
  K1 : Gain  Gain=-2*w_c*(1.0-lambda)/w_o  SaturateOnIntegerOverflow=on  OutDataTypeStr=Inherit: Same as input  ParamDataTypeStr=Inherit: Same as input
  K2 : Gain  Gain=2*w_o*(1.0-lambda)  SaturateOnIntegerOverflow=on  OutDataTypeStr=Inherit: Same as input  ParamDataTypeStr=Inherit: Same as input
  K3 : Gain  Gain=w_c  SaturateOnIntegerOverflow=on  OutDataTypeStr=Inherit: Same as input  ParamDataTypeStr=Inherit: Same as input
  K4 : Gain  Gain=K4  SaturateOnIntegerOverflow=on  OutDataTypeStr=Inherit: Same as input  ParamDataTypeStr=Inherit: Same as input
  LP filter : TransferFcn  Numerator=[w_c]  Denominator=[1 w_c]
  Notch filter : TransferFcn  Numerator=[1 2*zeta_n*w_o w_o*w_o]  Denominator=[1 2*w_o w_o^2]
  Sum{1,3..5} (4 alike) : Sum  Inputs=++|  InputSameDT=on  SaturateOnIntegerOverflow=on  OutDataTypeStr=Inherit: Same as first input
  Sum2 : Sum  Inputs=+|-  InputSameDT=on  SaturateOnIntegerOverflow=on  OutDataTypeStr=Inherit: Same as first input
  Sum6 : Sum  Inputs=+--  InputSameDT=on  SaturateOnIntegerOverflow=on  OutDataTypeStr=Inherit: Same as first input
  Sum7 : Sum  Inputs=|+-  InputSameDT=on  SaturateOnIntegerOverflow=on  OutDataTypeStr=Inherit: Same as first input
  "ssa " : $bdroot/Utilities/Math Operations/ssa  SystemSampleTime=-1  VariantActivationTime=update diagram  AllowFlexibleInterface=on  Latency=0  AutoFrameSizeCalculation=off
  "ssa  " : $bdroot/Utilities/Math Operations/ssa  SystemSampleTime=-1  VariantActivationTime=update diagram  AllowFlexibleInterface=on  Latency=0  AutoFrameSizeCalculation=off
  psi_w : Outport  VectorParamsAs1DForOutWhenUnconnected=off
  psi : Outport  Port=2  VectorParamsAs1DForOutWhenUnconnected=off
  r : Outport  Port=3  VectorParamsAs1DForOutWhenUnconnected=off
  wires:
  K4/1 -> Sum1/1
  Sum3/1 -> Integrator/1
  Sum2/1 -> "ssa  "/1
  "ssa  "/1 -> K1/1, K2/1, K3/1, Sum7/1
  Integrator/1 -> "ssa "/1  "psi"
  "ssa "/1 -> psi/1, Sum4/2
  Sum4/1 -> Sum2/2
  K3/1 -> Sum3/1
  Sum6/1 -> Integrator1/1
  Gain1/1 -> Sum6/3
  Gain2/1 -> Sum6/2
  Integrator2/1 -> Gain2/1  "xi_W"
  K1/1 -> Sum5/1
  K2/1 -> Sum6/1
  Sum5/1 -> Integrator2/1  "psi_WF"
  Integrator1/1 -> Sum5/2, Gain1/1, Sum4/1, psi_w/1  "psi_w"
  Integrator3/1 -> Gain3/1, K4/1  "bias"
  Notch filter/1 -> LP filter/1  "r_LF"
  Sum1/1 -> Notch filter/1
  LP filter/1 -> Sum3/2, r/1
  Sum7/1 -> Integrator3/1
  Gain3/1 -> Sum7/2
  compass/1 -> Sum2/1
  rate gyro/1 -> Sum1/2

== system mssSimulink/Utilities/Dynamics/2nd order time constant ==
  In : Inport
  Transfer Fcn1 : TransferFcn  Denominator=[1/(1.5/T)^2 2/(1.5/T) 1]
  Out : Outport  VectorParamsAs1DForOutWhenUnconnected=off
  wires:
  In/1 -> Transfer Fcn1/1
  Transfer Fcn1/1 -> Out/1

== system mssSimulink/Utilities/Math Operations/Unit Conversion ==
  In : Inport
  Gain : Gain  Gain=k  SaturateOnIntegerOverflow=on  OutDataTypeStr=Inherit: Same as input  ParamDataTypeStr=Inherit: Same as input
  Out : Outport  VectorParamsAs1DForOutWhenUnconnected=off
  wires:
  In/1 -> Gain/1
  Gain/1 -> Out/1

== system mssSimulink/Utilities/Math Operations/[-inf inf] to [-pi pi] ==
  note: r
  note: x
  x [-inf inf] : Inport
  Constant : Constant  Value=2*pi
  Gain : Gain  Gain=pi  SaturateOnIntegerOverflow=on  OutDataTypeStr=Inherit: Same as input  ParamDataTypeStr=Inherit: Same as input
  Math Function : Math  Operator=rem  SignedPower=on
  Saturation : Saturate  UpperLimit=1e10  LowerLimit=-1e10
  Sign : Signum
  Sum : Sum  Inputs=|+-  SaturateOnIntegerOverflow=on
  Sum1 : Sum  Inputs=|++  SaturateOnIntegerOverflow=on
  y [-pi pi] : Outport  VectorParamsAs1DForOutWhenUnconnected=off
  wires:
  Saturation/1 -> Sign/1, Sum1/1
  Sum/1 -> y [-pi pi]/1
  Math Function/1 -> Sum/1
  Constant/1 -> Math Function/2
  Sum1/1 -> Math Function/1
  Gain/1 -> Sum1/2, Sum/2
  Sign/1 -> Gain/1
  x [-inf inf]/1 -> Saturation/1

== system mssSimulink/Utilities/Math Operations/[-pi pi] to [-inf inf] ==
  x [-pi pi] : Inport
  S-Function : S-Function  FunctionName=pipi2inf  SFunctionDeploymentMode=off  EnableBusSupport=off
  y [-inf inf] : Outport  VectorParamsAs1DForOutWhenUnconnected=off
  wires:
  S-Function/1 -> y [-inf inf]/1
  x [-pi pi]/1 -> S-Function/1

== system mssSimulink/Utilities/Math Operations/deg to 180//180 ==
  note: r
  note: x
  x (deg) : Inport
  Constant : Constant  Value=2*180
  Gain : Gain  Gain=180  SaturateOnIntegerOverflow=on  OutDataTypeStr=Inherit: Same as input  ParamDataTypeStr=Inherit: Same as input
  Math Function : Math  Operator=rem  SignedPower=on
  Saturation : Saturate  UpperLimit=1e10  LowerLimit=-1e10
  Sign : Signum
  Sum : Sum  Inputs=|+-  SaturateOnIntegerOverflow=on
  Sum1 : Sum  Inputs=|++  SaturateOnIntegerOverflow=on
  -180<y<180 : Outport  VectorParamsAs1DForOutWhenUnconnected=off
  wires:
  Sum/1 -> -180<y<180/1
  Math Function/1 -> Sum/1
  Constant/1 -> Math Function/2
  Sum1/1 -> Math Function/1
  Gain/1 -> Sum1/2, Sum/2
  Sign/1 -> Gain/1
  x (deg)/1 -> Saturation/1
  Saturation/1 -> Sign/1, Sum1/1

== system mssSimulink/Utilities/Math Operations/ssa ==
  angle : Inport
  " " : Math  Operator=mod
  Constant : Constant  Value=2*pi
  Constant1 : Constant  Value=pi
  Sum : Sum  Inputs=|++
  Sum1 : Sum  Inputs=-+|
  angle_pipi : Outport
  wires:
  angle/1 -> Sum/2
  Constant/1 -> " "/2
  Sum1/1 -> angle_pipi/1
  " "/1 -> Sum1/2
  Constant1/1 -> Sum1/1, Sum/1
  Sum/1 -> " "/1

== system mssSimulink/Utilities/Simulation tools/6DOF comparison ==
  In 1 : Inport
  In 2 : Inport  Port=2
  6DOF comparison : Scope  NumInputPorts=6
  Demux1 : Demux  Outputs=6
      settings: DisplayOption=none
  Demux2 : Demux  Outputs=6
      settings: DisplayOption=none
  Mux{,1..5} (6 alike) : Mux  Inputs=2
  wires:
  Demux2/1 -> Mux/1  "surge"
  Demux1/1 -> Mux/2  "surge"
  Demux2/2 -> Mux1/1  "sway"
  Demux2/3 -> Mux2/1  "heave"
  Demux2/4 -> Mux3/1  "roll"
  Demux2/5 -> Mux4/1  "pitch"
  Demux2/6 -> Mux5/1  "yaw"
  Demux1/2 -> Mux1/2
  Demux1/3 -> Mux2/2
  Demux1/4 -> Mux3/2
  Demux1/5 -> Mux4/2
  Demux1/6 -> Mux5/2
  In 1/1 -> Demux2/1
  In 2/1 -> Demux1/1
  Mux/1 -> 6DOF comparison/1  "surge"
  Mux1/1 -> 6DOF comparison/2  "sway"
  Mux2/1 -> 6DOF comparison/3  "heave"
  Mux3/1 -> 6DOF comparison/4  "roll"
  Mux4/1 -> 6DOF comparison/5  "pitch"
  Mux5/1 -> 6DOF comparison/6  "yaw"

== system mssSimulink/Utilities/Simulation tools/Signal range error ==
  Signal : Inport
  Add : Sum
  Constant : Constant  Value=Values
  MinMax : MinMax  Function=max
  MinMax1 : MinMax  Function=max
  MinMax2 : MinMax
  MinMax3 : MinMax
  Saturation : Saturate  UpperLimit=1  LowerLimit=0
  Saturation1 : Saturate  UpperLimit=1  LowerLimit=0
  Sign : Signum
  Sign1 : Signum
  Stop simulation : $bdroot/Utilities/Simulation tools/Stop simulation  message=message
  Subtract : Sum  Inputs=+-
  Subtract1 : Sum  Inputs=-+
  wires:
  Sign/1 -> Saturation/1
  Signal/1 -> MinMax/1, MinMax2/1
  Constant/1 -> MinMax1/1, MinMax3/1
  MinMax/1 -> Subtract/1
  MinMax1/1 -> Subtract/2
  Subtract/1 -> Sign/1
  Saturation/1 -> Add/1
  Add/1 -> Stop simulation/1
  Sign1/1 -> Saturation1/1
  Subtract1/1 -> Sign1/1
  MinMax2/1 -> Subtract1/1
  MinMax3/1 -> Subtract1/2
  Saturation1/1 -> Add/2

== system mssSimulink/Utilities/Visualization/North-East plot ==
  xpos : Inport
  ypos : Inport  Port=2
  wptX : Inport  Port=3
  wptY : Inport  Port=4
  Mux : Mux  Inputs=2
  To Workspace : ToWorkspace  VariableName=xyplot  SaveFormat=Timeseries  SampleTime=-1
      settings: Decimation=decimation
  To Workspace1 : ToWorkspace  VariableName=waypoints  SampleTime=-1
      settings: Save2DSignal=2-D array (concatenate along first dimension)
  Vector Concatenate : Concatenate  Mode=Multidimensional array  ConcatenateDimension=2
  wires:
  ypos/1 -> Mux/2
  xpos/1 -> Mux/1
  Mux/1 -> To Workspace/1
  wptX/1 -> Vector Concatenate/1
  wptY/1 -> Vector Concatenate/2
  Vector Concatenate/1 -> To Workspace1/1

== system mssSimulink/Utilities/Visualization/North-East plot   ==
  xpos : Inport
  ypos : Inport  Port=2
  Mux : Mux  Inputs=2
  To Workspace : ToWorkspace  VariableName=xyplot  SaveFormat=Timeseries  SampleTime=-1
      settings: Decimation=100
  wires:
  ypos/1 -> Mux/2
  xpos/1 -> Mux/1
  Mux/1 -> To Workspace/1

== system mssSimulink/Environment/Wind/Isherwood (1972) wind forces/If gamm_r > 0 then feedthrough ==
  6 DOF : Inport
  Action Port : ActionPort
  "6 DOF  " : Outport  VectorParamsAs1DForOutWhenUnconnected=off
  wires:
  6 DOF/1 -> "6 DOF  "/1

== system mssSimulink/Environment/Wind/Isherwood (1972) wind forces/If gamma_r <0 then change sign ==
  6 DOF : Inport
  Action Port : ActionPort
  Constant : Constant  Value=[1 -1 1 -1 1 -1]
  Product : Product  SaturateOnIntegerOverflow=on  OutDataTypeStr=Inherit: Same as first input
  "6 DOF  " : Outport  VectorParamsAs1DForOutWhenUnconnected=off
  wires:
  6 DOF/1 -> Product/1
  Product/1 -> "6 DOF  "/1
  Constant/1 -> Product/2

== system mssSimulink/Environment/Wind/Wind/Slowly-varying wind ==
  Enable : EnablePort
  Band-Limited White Noise : simulink/Sources/Band-Limited White Noise  Cov=Par_Wind_speed_noise_pow  Ts=Par_Wind_sample_time  seed=Par_Wind_speed_seed
  "Band-Limited White Noise " : simulink/Sources/Band-Limited White Noise  Cov=Par_Wind_angle_noise_pow  Ts=Par_Wind_sample_time  seed=Par_Wind_angle_seed
  Gain : Gain  Gain=1/Par_Wind_speed_T  SaturateOnIntegerOverflow=on  OutDataTypeStr=Inherit: Same as input  ParamDataTypeStr=Inherit: Same as input
  "Gain " : Gain  Gain=1/Par_Wind_angle_T  SaturateOnIntegerOverflow=on  OutDataTypeStr=Inherit: Same as input  ParamDataTypeStr=Inherit: Same as input
  Integrator : Integrator  LimitOutput=on  UpperSaturationLimit=Par_Wind_speed_rand_max  LowerSaturationLimit=-Par_Wind_speed_rand_max
  "Integrator " : Integrator  LimitOutput=on  UpperSaturationLimit=Par_Wind_angle_rand_max  LowerSaturationLimit=-Par_Wind_angle_rand_max
  Sum : Sum  Inputs=|+-  InputSameDT=on  SaturateOnIntegerOverflow=on  OutDataTypeStr=Inherit: Same as first input
  "Sum       " : Sum  Inputs=|+-  InputSameDT=on  SaturateOnIntegerOverflow=on  OutDataTypeStr=Inherit: Same as first input
  angle : Outport  InitialOutput=0  VectorParamsAs1DForOutWhenUnconnected=off
  speed : Outport  Port=2  InitialOutput=0  VectorParamsAs1DForOutWhenUnconnected=off
  wires:
  Band-Limited White Noise/1 -> Sum/1
  Integrator/1 -> Sum/2, speed/1
  Sum/1 -> Gain/1
  Gain/1 -> Integrator/1
  "Band-Limited White Noise "/1 -> "Sum       "/1
  "Integrator "/1 -> "Sum       "/2, angle/1
  "Sum       "/1 -> "Gain "/1
  "Gain "/1 -> "Integrator "/1

== system mssSimulink/Environment/Wind/Wind/Wind gust ==
  u10 : Inport
  Enable : EnablePort
  Clock : Clock
  Dot Product : DotProduct  OutDataTypeStr=Inherit: Inherit via internal rule
  Frequencies : Constant  Value=Par_Wind_minfreq:(Par_Wind_maxfreq - Par_Wind_minfreq)/(Par_Wind_nfreq-1):Par_Wind_maxfreq
  Gain : Gain  Gain=2  SaturateOnIntegerOverflow=on  OutDataTypeStr=Inherit: Same as input  ParamDataTypeStr=Inherit: Same as input
  Gain1 : Gain  Gain=2*pi  SaturateOnIntegerOverflow=on  OutDataTypeStr=Inherit: Same as input  ParamDataTypeStr=Inherit: Same as input
  Harris spectrum : Subsystem
  Math Function1 : Math  Operator=sqrt  SignedPower=on
  Multiport Switch : MultiPortSwitch  Inputs=2  RndMeth=Nearest  InputSameDT=off
  NORSOK spectrum : Subsystem
  Phase generator : Subsystem
  Product1 : Product  SaturateOnIntegerOverflow=on  OutDataTypeStr=Inherit: Same as first input
  Product2 : Product  SaturateOnIntegerOverflow=on  OutDataTypeStr=Inherit: Same as first input
  Saturation : Saturate  UpperLimit=2  LowerLimit=1
  Spectrum type : Constant  Value=Par_Wind_spectrum_type
  Sum : Sum  SaturateOnIntegerOverflow=on
  Trigonometric Function : Trigonometry
  dfreq : Constant  Value=(Par_Wind_maxfreq - Par_Wind_minfreq)/(Par_Wind_nfreq -1)
  Gust : Outport  InitialOutput=0  VectorParamsAs1DForOutWhenUnconnected=off
  wires:
  Saturation/1 -> Multiport Switch/1
  Frequencies/1 -> Harris spectrum/1(Freqs), NORSOK spectrum/1(Freqs), Gain1/1
  u10/1 -> NORSOK spectrum/2(u10), Harris spectrum/2(u10)
  Gain/1 -> Product1/1
  dfreq/1 -> Product1/2
  Product1/1 -> Math Function1/1
  Multiport Switch/1 -> Gain/1
  Spectrum type/1 -> Saturation/1
  Harris spectrum/1(S) -> Multiport Switch/2
  NORSOK spectrum/1(S) -> Multiport Switch/3
  Gain1/1 -> Product2/1
  Clock/1 -> Product2/2, Phase generator/Trigger
  Product2/1 -> Sum/1  "wt"
  Phase generator/1(Phase) -> Sum/2
  Sum/1 -> Trigonometric Function/1
  Math Function1/1 -> Dot Product/1  "Amp"
  Trigonometric Function/1 -> Dot Product/2  "sin(wt + phase)"
  Dot Product/1 -> Gust/1

== system mssSimulink/Guidance/Waypoint guidance block/Stop vessel/Reached endpoint ==
  IfAction : ActionPort
  Constant : Constant  Value=0
  Stop Simulation : Stop
  stop : Constant  Value=stop
  zero : Outport  VectorParamsAs1DForOutWhenUnconnected=off
  wires:
  Constant/1 -> zero/1
  stop/1 -> Stop Simulation/1

== system mssSimulink/Guidance/Waypoint guidance block/Stop vessel/Still travelling ==
  IfAction : ActionPort
  Constant : Constant
  one : Outport  VectorParamsAs1DForOutWhenUnconnected=off
  wires:
  Constant/1 -> one/1

== system mssSimulink/Guidance/Waypoint guidance block/Thetacomputation/5th order algorithm ==
  theta : Inport
  IfAction : ActionPort
  Constant1 : Constant
  Constant2 : Constant
  Math Function : Math  Operator=mod  SignedPower=on
  Mux1 : Mux  Inputs=6
  Product{,1..3} (4 alike) : Product  InputSameDT=on  SaturateOnIntegerOverflow=on  OutDataTypeStr=Inherit: Same as first input
  theta_vector : Outport  VectorParamsAs1DForOutWhenUnconnected=off
  wires:
  Constant1/1 -> Math Function/2
  Math Function/1 -> Product/1, Product1/2, Product2/2, Product3/2, Mux1/5, Product/2
  theta/1 -> Math Function/1
  Product/1 -> Product1/1, Mux1/4  "t^2"
  Product1/1 -> Product2/1, Mux1/3  "t^3"
  Product2/1 -> Mux1/2, Product3/1  "t^4"
  Product3/1 -> Mux1/1
  Constant2/1 -> Mux1/6
  Mux1/1 -> theta_vector/1

== system mssSimulink/Guidance/Waypoint guidance block/Thetacomputation/Cubic splines ==
  theta : Inport
  IfAction : ActionPort
  Constant1 : Constant
  Constant2 : Constant  Value=0
  Mux1 : Mux  Inputs=6
  Product : Product  InputSameDT=on  SaturateOnIntegerOverflow=on  OutDataTypeStr=Inherit: Same as first input
  Product1 : Product  InputSameDT=on  SaturateOnIntegerOverflow=on  OutDataTypeStr=Inherit: Same as first input
  theta_vector : Outport  VectorParamsAs1DForOutWhenUnconnected=off
  wires:
  theta/1 -> Product/1, Product/2, Product1/2, Mux1/3
  Product/1 -> Product1/1, Mux1/2  "t^2"
  Mux1/1 -> theta_vector/1
  Product1/1 -> Mux1/1  "t^3"
  Constant1/1 -> Mux1/4
  Constant2/1 -> Mux1/5, Mux1/6

== system mssSimulink/Guidance/Waypoint guidance block/vs_calculations/vs_calc ==
  ud : Inport
  xd_theta : Inport  Port=2
  yd_theta : Inport  Port=3
  Math Function : Math  Operator=square  SignedPower=on
  Math Function1 : Math  Operator=square  SignedPower=on
  Math Function2 : Math  Operator=sqrt  SignedPower=on
  Product : Product  Inputs=*/  InputSameDT=on  SaturateOnIntegerOverflow=on  OutDataTypeStr=Inherit: Same as first input
  Sum : Sum  Inputs=|++  InputSameDT=on  SaturateOnIntegerOverflow=on  OutDataTypeStr=Inherit: Same as first input
  vs : Outport  VectorParamsAs1DForOutWhenUnconnected=off
  wires:
  Math Function/1 -> Sum/1
  Math Function1/1 -> Sum/2
  Sum/1 -> Math Function2/1
  Math Function2/1 -> Product/2
  xd_theta/1 -> Math Function/1
  ud/1 -> Product/1
  Product/1 -> vs/1  "vs"
  yd_theta/1 -> Math Function1/1

== system mssSimulink/Guidance/Waypoint guidance block/vs_calculations/vs_t_calc ==
  xd_theta : Inport
  yd_theta : Inport  Port=2
  ud_dot : Inport  Port=3
  Math Function3 : Math  Operator=square  SignedPower=on
  Math Function4 : Math  Operator=square  SignedPower=on
  Math Function5 : Math  Operator=sqrt  SignedPower=on
  Product7 : Product  Inputs=*/  InputSameDT=on  SaturateOnIntegerOverflow=on  OutDataTypeStr=Inherit: Same as first input
  Sum3 : Sum  Inputs=|++  InputSameDT=on  SaturateOnIntegerOverflow=on  OutDataTypeStr=Inherit: Same as first input
  vs_t : Outport  VectorParamsAs1DForOutWhenUnconnected=off
  wires:
  xd_theta/1 -> Math Function3/1
  yd_theta/1 -> Math Function4/1
  Math Function3/1 -> Sum3/1
  Math Function4/1 -> Sum3/2
  Sum3/1 -> Math Function5/1
  Math Function5/1 -> Product7/2
  ud_dot/1 -> Product7/1
  Product7/1 -> vs_t/1
